simulink subsystem "theta_Offset_Calc"  (R2025b)
settings: Solver=VariableStepAuto
settings Model: Creator=kara  LastModifiedBy=Cheng
settings RTWCC: GPUComputeCapability=3.5

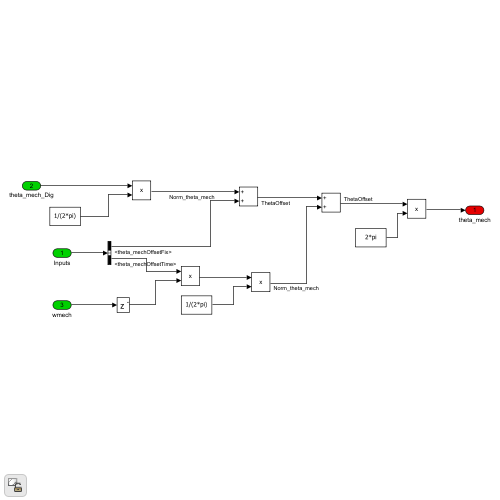
[thumbnail: Simulink's stored preview of the top-level diagram]
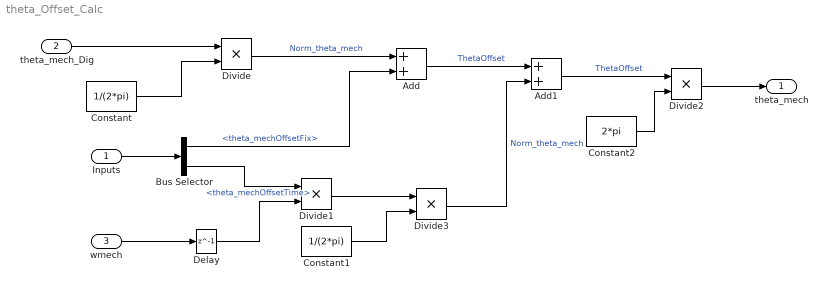
== system theta_Offset_Calc ==
  Inputs : Inport
  theta_mech_Dig : Inport  Port=2
  wmech : Inport  Port=3
  Add : Sum
  Add1 : Sum
  Bus Selector : BusSelector  OutputSignals=ControlParameter.Offsets.theta_mechOffsetFix,ControlParameter.Offsets.theta_mechOffsetTime
  Constant : Constant  Value=1/(2*pi)  OutDataTypeStr=PWMGenSacling
  Constant1 : Constant  Value=1/(2*pi)  OutDataTypeStr=PWMGenSacling
  Constant2 : Constant  Value=2*pi  OutDataTypeStr=UHighScaling
  Delay : Delay  DelayLength=1
  Divide : Product  Inputs=**  OutDataTypeStr=fixdt(0,32,32)
  Divide1 : Product  Inputs=**  OutDataTypeStr=HighScaling
  Divide2 : Product  Inputs=**  OutDataTypeStr=HighScaling
  Divide3 : Product  Inputs=**  OutDataTypeStr=fixdt(0,32,32)
  theta_mech : Outport
  wires:
  Constant2/1 -> Divide2/2
  Add1/1 -> Divide2/1  "ThetaOffset"
  theta_mech_Dig/1 -> Divide/1
  Divide/1 -> Add/1  "Norm_theta_mech"
  Constant/1 -> Divide/2
  Add/1 -> Add1/1  "ThetaOffset"
  Inputs/1 -> Bus Selector/1
  Bus Selector/1 -> Add/2  "<theta_mechOffsetFix>"
  Bus Selector/2 -> Divide1/1  "<theta_mechOffsetTime>"
  wmech/1 -> Delay/1
  Divide1/1 -> Divide3/1
  Constant1/1 -> Divide3/2
  Divide3/1 -> Add1/2  "Norm_theta_mech"
  Delay/1 -> Divide1/2
  Divide2/1 -> theta_mech/1
